simulink model "DP_STD_MDL_Boost_2022b"  (R2022b)
settings: Solver=VariableStepAuto  StartTime=0.0  StopTime=0.1  RelTol=1e-3
libraries: spsSeriesRLCBranchLib x4, spsMosfetLib x2, peripheral_utilities x2, spsCurrentMeasurementLib x1, spsSecondOrderFilterLib x1, spsVoltageMeasurementLib x1, spsControlledVoltageSourceLib x1, gmp_sil_core_pack x1, spsGroundLib x1, spspowerguiLib x1
settings Model: Creator=javnson  LastModifiedBy=javnson
settings OptimizationCC: ReuseModelBlockBuffer=on
settings RTWCC: GPUComputeCapability=5.0

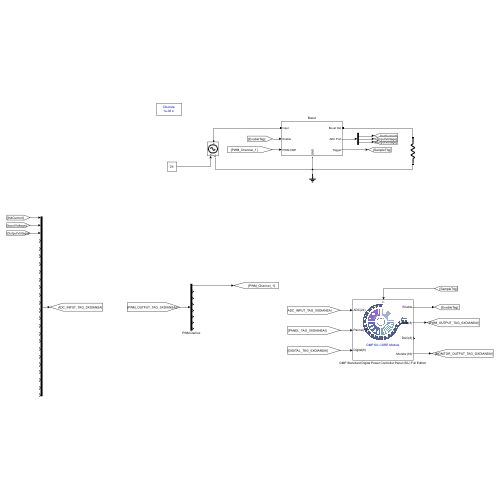
[thumbnail: Simulink's stored preview of the top-level diagram]
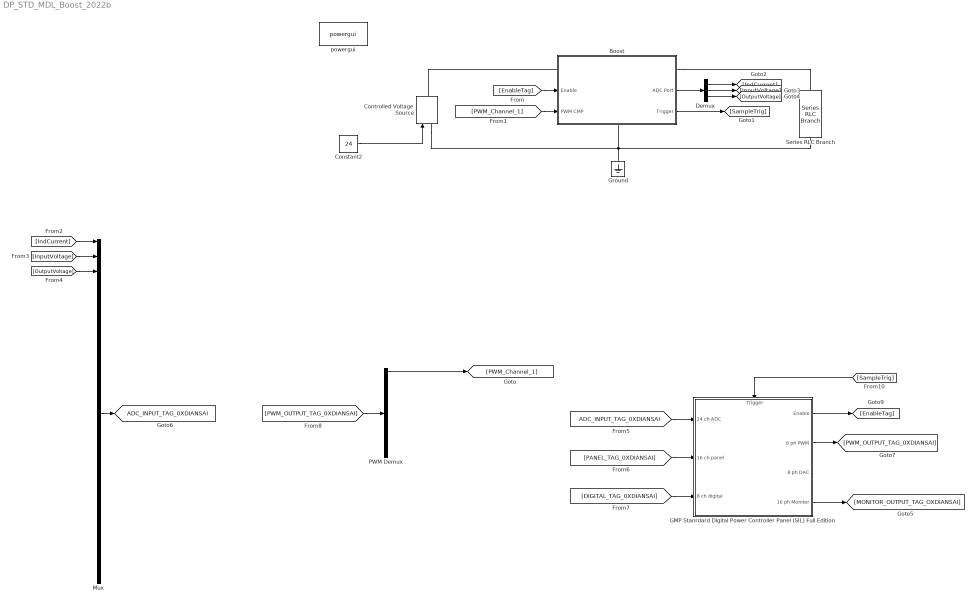
== system DP_STD_MDL_Boost_2022b ==
  Boost : Subsystem  mask(GMP Standard Digital Power Submodule - Boost){R_mosfet_on=4.6e-3, Lon=0, Rd=0.01, Vf=0.5, Rs=1e5, Cs=inf, L_main=1e-3, L_ESR=15e-3, Cin_main=100e-6, Cin_ESR=1.5, Cout_main=100e-6, Cout_ESR=1.5, fswitch=20e3, CMP_MAX=5000, Deadband_Upper=50, Deadband_Lower=50, phase_shift=0, ADC_Resolution=12, Voltage_Gain=1, VOLTAGE_ADC_REFERENCE=80, VOLTAGE_ADC_BIAS=40, VOLTAGE_ADC_INIT=0, VOLTAGE_ADC_CUT_FREQ=1.5e3, Current_Gain=1, CURRENT_ADC_REFERENCE=10, CURRENT_ADC_BIAS=5, CURRENT_ADC_INIT=0}
      mask prompts: ADC_Resolution "ADC_BIT:"; Voltage_Gain "ADC_GAIN:"; VOLTAGE_ADC_REFERENCE "ADC_REFERENCE:"; VOLTAGE_ADC_BIAS "ADC_BIAS:"; VOLTAGE_ADC_INIT "ADC_INIT:"; VOLTAGE_ADC_CUT_FREQ "cut_frequency:"; Current_Gain "ADC_GAIN:"; CURRENT_ADC_REFERENCE "ADC_REFERENCE:"; CURRENT_ADC_BIAS "ADC_BIAS:"; CURRENT_ADC_INIT "ADC_INIT:"
      mask help: This is a Standard Boost Module.
      settings: PortSchema="{\"entries\":[{\"content\":{\"sides\":[{\"content\":{\"connectorIds\":[\"LConn1\",\"In1\",\"In2\"]},\"type\":\"ConnectorPlacement.EquallySpacedRectSide\",\"uuid\":\"14f7e26c-4d08-496b-8d9c-39acdf23712e\"},{\"content\":{\"connectorIds\":[\"RConn1\",\"Out1\",\"Out2\"],\"side\":\"RIGHT\"},\"type\":\"ConnectorPlacement.EquallySpacedRectSide\",\"uuid\":\"c4fec36d-dc89-4255-810a-778c215f41bb\"},{\"content\":{\"side\":\"TOP\"},\"type\":\"ConnectorPlacement.EquallySpacedRectSide\",\"uuid\":\"1b2864bd-03e2-4902-8158-79673144629a\"},{\"content\":{\"connectorIds\":[\"RConn2\"],\"side\":\"BOTTOM\"},\"type\":\"ConnectorPlacement.EquallySpacedRectSide\",\"uuid\":\"d3456d19-e299-4c35-abfd-6fb99773e971\"}]},\"type\":\"ConnectorPlacement.EquallySpacedConnector\",\"uuid\":\"dbc738c4-c361-40e9-b3e6-9b32447065a0\"}],\"packageUris\":[\"http://schema.mathworks.com/mf0/Connector/R2020b\"],\"version\":\"1.0\"}"
      mask DialogControl ParameterGroupVar Prompt: 参数
      mask DialogControl Container4 Prompt: Component Parameters
      mask DialogControl Container7 Prompt: MOSFET
      mask DialogControl Control8 Prompt: Rds(on), unit Ohm
      mask DialogControl Control9 Prompt: Internal diode inducctance, unit H
      mask DialogControl Control10 Prompt: Internal diode resistance Rd, unit Ohm
      mask DialogControl Control11 Prompt: Internal diode forward voltage Vf, unit V
      mask DialogControl Control12 Prompt: Snubber resistance Rs, unit ohm
      mask DialogControl Control13 Prompt: Snubber Capacitance Cs, unit F
      mask DialogControl Container8 Prompt: LC Filter
      mask DialogControl Control25 Prompt: main inductance (H):
      mask DialogControl Control26 Prompt: Inductance ESR (Ohm):
      mask DialogControl Control27 Prompt: Main Input Capacitor (F):
      mask DialogControl Control28 Prompt: Input Capcitor ESR (Ohm):
      mask DialogControl Control29 Prompt: Main Output Capacitor (F):
      mask DialogControl Control30 Prompt: Output Capcitor ESR (Ohm):
      mask DialogControl Container5 Prompt: PWM Parameers
      mask DialogControl Control3 Prompt: PWM Frequency (Hz):
      mask DialogControl Control4 Prompt: Full Scale PWM Compare value:
      mask DialogControl Control6 Prompt: (whole period is 2 * CMP_MAX ticks)
      mask DialogControl Control5 Prompt: Deadband Range Set (CMP Value):
      mask DialogControl Control7 Prompt: Single side deadband time: DEADBAND_CMP/2/CMP_MAX/fswitch
      mask DialogControl Control2 Prompt: Initial Phase Shift, unit rad
      mask DialogControl Container6 Prompt: ADC Parameters
      mask DialogControl Container9 Prompt: ADC Device
      mask DialogControl Control14 Prompt: ADC resolution:
      mask DialogControl Container10 Prompt: Voltage Sensor
      mask DialogControl Control15 Prompt: ADC Voltage Gain (Scale Factor):
      mask DialogControl Control16 Prompt: ADC reference Voltage(V)
      mask DialogControl Control Prompt: ADC Bias Voltage(V)
      mask DialogControl Control18 Prompt: ADC Initial Voltage Output (V):
      mask DialogControl Control19 Prompt: Voltage Filter cut frequency (Hz):
      mask DialogControl Control20 Prompt: Generally, this value less than switch frequency / 10, greater than motor normal frequency * 3
      mask DialogControl Container11 Prompt: Current Sensor
      mask DialogControl Control21 Prompt: ADC Current Gain (Scale Factor):
      mask DialogControl Control22 Prompt: ADC reference Current(A), ADC full scale current (when gain = 1)
      mask DialogControl Control23 Prompt: ADC Bias Current(A)
      mask DialogControl Control24 Prompt: ADC initial Current Output(A)
  Constant2 : Constant  Value=24
  Controlled Voltage Source : spsControlledVoltageSourceLib/Controlled Voltage Source  Initialize=on  Source_Type=AC  Amplitude=0  Phase=0  Frequency=0  Measurements=None
  Demux : Demux  Outputs=3
  GMP Stanrdard Digital Power Controller Panel (SIL) Full Edition : Subsystem  mask(GMP SIL Core for single Motor Controller (full edition)){}
      mask help: This is GMP Motor Simulator port.
      settings: PortSchema="{\"entries\":[{\"content\":{\"sides\":[{\"content\":{\"connectorIds\":[\"In1\",\"In2\",\"In3\"]},\"type\":\"ConnectorPlacement.EquallySpacedRectSide\",\"uuid\":\"45c67bc9-9540-469a-a4ac-1e12eb9acca3\"},{\"content\":{\"connectorIds\":[\"Out1\",\"Out2\",\"Out3\",\"Out4\"],\"side\":\"RIGHT\"},\"type\":\"ConnectorPlacement.EquallySpacedRectSide\",\"uuid\":\"a17116b4-0460-48ab-8ada-a785da6c5e29\"},{\"content\":{\"connectorIds\":[\"In4\"],\"side\":\"TOP\"},\"type\":\"ConnectorPlacement.EquallySpacedRectSide\",\"uuid\":\"15623697-512e-4e4d-ab51-f53c2346fadb\"},{\"content\":{\"side\":\"BOTTOM\"},\"type\":\"ConnectorPlacement.EquallySpacedRectSide\",\"uuid\":\"47f7968c-22c1-4f3d-97d9-242e9dbf8d30\"}]},\"type\":\"ConnectorPlacement.EquallySpacedConnector\",\"uuid\":\"f369880c-e675-4c1f-982e-a4befb03f503\"}],\"packageUris\":[\"http://schema.mathworks.com/mf0/Connector/R2020b\"],\"version\":\"1.0\"}"
      mask DialogControl ParameterGroupVar Prompt: 参数
      mask Display:
      | image(append(fileparts(which('gmp_simulink_utilities.slx')),'\icon\GMP_Core.png'));
      | color('blue');
      | %text(0.3,0.3,'GMP SIL CORE Module','horizontalAlignment','left','verticalAlignment','bottom');
      | disp('\n\n\n\n\n\n\n\nGMP SIL CORE Module');
      | %text(0,0,'y=a*x^2+b','horizontalAlignment','middle', 'verticalAlignment','bottom');
      | 
      | 
      | module_pos = get_param(gcb, 'Position');
      | width = module_pos(3) - module_pos(1);
      | %rectangle('Position',[module_pos(1),module_pos(2),module_pos(3),module_pos(4)],'FaceColor','r');
      | 
      | color('Black');
      | 
      | port_label('output', 1, 'Enable');
      | port_label('output', 2, 'PWM(8)');
      | port_label('output', 3, 'DAC(8)');
      | port_label('output', 4, 'Monitor(16)');
      | 
      | port_label('input', 1, 'ADC(24)');
      | port_label('input', 2, 'Pannel(16)');
      | port_label('input', 3, 'Digital(8)');
      | port_label('input', 4, 'T');
  Ground : spsGroundLib/Ground  LConnTagsString=a
  Mux : Mux  Inputs=24
  PWM Demux : Demux  Outputs=8
  Series RLC Branch : spsSeriesRLCBranchLib/Series RLC Branch  LConnTagsString=__new0  RConnTagsString=__new0  BranchType=R  Resistance=10  Inductance=1e-3  SetiL0=off  InitialCurrent=0  Capacitance=1e-6  Setx0=off  InitialVoltage=0  Measurements=None
  powergui : spspowerguiLib/powergui  Priority=1  SimulationMode=Discrete  SampleTime=1e-6  frequency=60  Iterations=50  frequencyindice=0  Pbase=100e6  ErrMax=1e-4  UnitsV=kV  UnitsW=MW  buscounter=0  FunctionMessages=off  echomessages=off  EnableUseOfTLC=off  CurrentSourceSwitches=off  DisableSnubberDevices=off  DisableRonSwitches=off  DisableVfSwitches=off  DisplayEquations=off  AutomaticDiscreteSolvers=off  SolverType=Tustin/Backward Euler (TBE)  Interpol=off  ExternalGateDelay=off  methode=off  Ts=100  x0status=blocks  SPID=on  SwTol=0  HookPort=off  NonlinearTolerance=1e-4  nMaxIteration=100  ContinueOnMaxIteration=off  RestoreLinks=warning  ResistiveCurrentMeasurement=off  Frange=[0:2:500]  Ylog=off  Xlog=on  ShowGrid=off  save=off  variable=ZData  structure=0  ZoomFFT=off  StartTime=0.0  cycles=1  DisplayStyle=1  fundamental=60  FreqAxis=off  MaxFrequency=1000  frequencyindicesteady=1  RmsSteady=1  display=off
  tag scope: ADC_INPUT_TAG_0XDIANSAI=global
  wires:
  [PWM_Channel_1] -> Boost/2(PWM CMP)
  Boost/1(ADC Port) -> Demux/1
  Demux/2 -> [InputVoltage]
  Demux/1 -> [IndCurrent]
  Demux/3 -> [OutputVoltage]
  Constant2/1 -> Controlled Voltage Source/1
  [SampleTrig] -> GMP Stanrdard Digital Power Controller Panel (SIL) Full Edition/4(Trigger)
  GMP Stanrdard Digital Power Controller Panel (SIL) Full Edition/1(Enable) -> [EnableTag]
  [EnableTag] -> Boost/1(Enable)
  PWM Demux/1 -> [PWM_Channel_1]
  Boost/2(Trigger) -> [SampleTrig]
  [IndCurrent] -> Mux/1
  [InputVoltage] -> Mux/2
  [OutputVoltage] -> Mux/3
  Mux/1 -> [ADC_INPUT_TAG_0XDIANSAI]
  [ADC_INPUT_TAG_0XDIANSAI] -> GMP Stanrdard Digital Power Controller Panel (SIL) Full Edition/1(24 ch ADC)
  [PANEL_TAG_0XDIANSAI] -> GMP Stanrdard Digital Power Controller Panel (SIL) Full Edition/2(16 ch panel)
  [DIGITAL_TAG_0XDIANSAI] -> GMP Stanrdard Digital Power Controller Panel (SIL) Full Edition/3(8 ch digital)
  [PWM_OUTPUT_TAG_0XDIANSAI] -> PWM Demux/1
  GMP Stanrdard Digital Power Controller Panel (SIL) Full Edition/2(8 ph PWM) -> [PWM_OUTPUT_TAG_0XDIANSAI]
  GMP Stanrdard Digital Power Controller Panel (SIL) Full Edition/4(16 ph Monitor) -> [MONITOR_OUTPUT_TAG_OXDIANSAI]
  connections:
  Controlled Voltage Source/RConn1 -- Boost/LConn1
  Controlled Voltage Source/LConn1 -- Series RLC Branch/RConn1 -- Ground/LConn1 -- Boost/RConn2
  Boost/RConn1 -- Series RLC Branch/LConn1

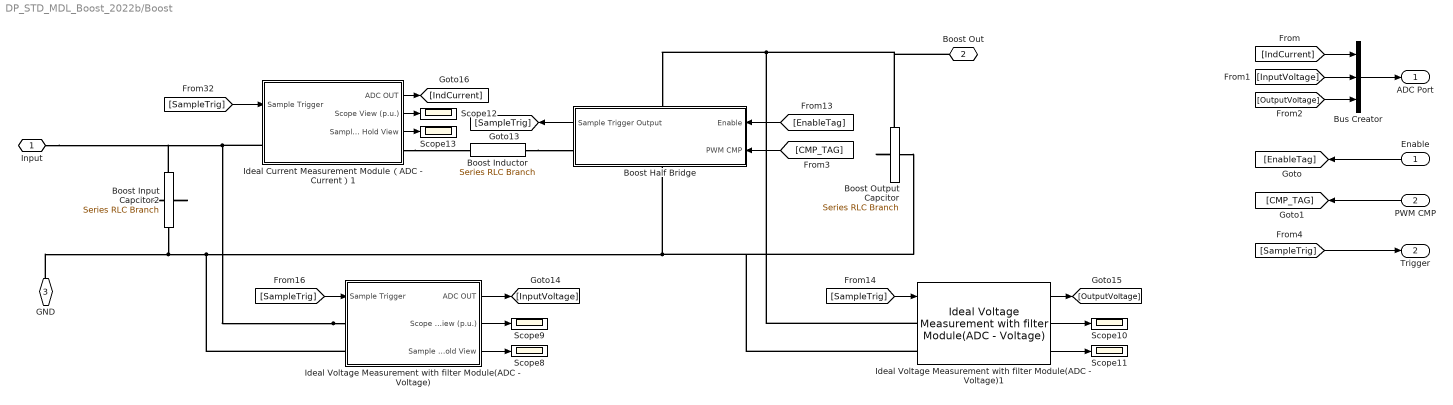
== system DP_STD_MDL_Boost_2022b/Boost ==
  Enable : Inport
  PWM CMP : Inport  Port=2
  Boost Half Bridge : Subsystem  AncestorBlock=peripheral_utilities/Single Phase Full Bridge  mask{fswitch=fswitch, CMP_MAX=CMP_MAX, Deadband_Upper=Deadband_Upper, Deadband_Lower=Deadband_Lower, Deadband_us=NaN, phase_shift=phase_shift, R_mosfet_on=R_mosfet_on, Lon=Lon, Rd=Rd, Vf=Vf, Rs=Rs, Cs=Cs}
      mask init:
      | calculate_deadband(gcb, 'Deadband_Upper', 'Deadband_Lower',	'CMP_MAX', 'fswitch', 'Deadband_us');
      settings: PortSchema="{\"entries\":[{\"content\":{\"sides\":[{\"content\":{\"connectorIds\":[\"In1\",\"In2\"]},\"type\":\"ConnectorPlacement.EquallySpacedRectSide\",\"uuid\":\"20beeabc-b0ca-4337-b227-c7f02abd15d8\"},{\"content\":{\"connectorIds\":[\"Out1\",\"RConn1\"],\"side\":\"RIGHT\"},\"type\":\"ConnectorPlacement.EquallySpacedRectSide\",\"uuid\":\"a7923383-ac55-4621-ad1d-4d067c1fb84d\"},{\"content\":{\"connectorIds\":[\"LConn1\"],\"side\":\"TOP\"},\"type\":\"ConnectorPlacement.EquallySpacedRectSide\",\"uuid\":\"661bf0ae-1c96-4de8-96aa-28c06a0a56db\"},{\"content\":{\"connectorIds\":[\"RConn2\"],\"side\":\"BOTTOM\"},\"type\":\"ConnectorPlacement.EquallySpacedRectSide\",\"uuid\":\"fc2f6321-5787-4e1a-b5a2-65ed34db36b5\"}]},\"type\":\"ConnectorPlacement.EquallySpacedConnector\",\"uuid\":\"e2219b16-0a50-43ef-8183-c55a35d5a2a0\"}],\"packageUris\":[\"http://schema.mathworks.com/mf0/Connector/R2020b\"],\"version\":\"1.0\"}"
      mask Callback fswitch: calculate_deadband(gcb, 'Deadband_Upper', 'Deadband_Lower',	'CMP_MAX', 'fswitch', 'Deadband_us');
      mask Callback CMP_MAX: calculate_deadband(gcb, 'Deadband_Upper', 'Deadband_Lower',	'CMP_MAX', 'fswitch', 'Deadband_us');
      mask Callback Deadband_Upper: calculate_deadband(gcb, 'Deadband_Upper', 'Deadband_Lower',	'CMP_MAX', 'fswitch', 'Deadband_us');
      mask Callback Deadband_Lower: calculate_deadband(gcb, 'Deadband_Upper', 'Deadband_Lower',	'CMP_MAX', 'fswitch', 'Deadband_us');
      mask DialogControl DescGroupVar Prompt: Half Bridge With PWM Module
      mask DialogControl Control14 Prompt: GMP CTL Simulink Utilities: virtual peripherals
      mask DialogControl DescTextVar Prompt: This module provide a PWM (with deadband), and a MOSFET half bridge.
      mask DialogControl Container5 Prompt: PWM Modulator
      mask DialogControl ParameterGroupVar Prompt: PWM module parameters
      mask DialogControl Control2 Prompt: PWM Frequency (Hz):
      mask DialogControl Control3 Prompt: Full Scale PWM Compare value:
      mask DialogControl Control4 Prompt: (whole period is 2 * CMP_MAX ticks)
      mask DialogControl Control5 Prompt: Deadband Range Set (CMP Value):
      mask DialogControl Control6 Prompt: Single side deadband time: DEADBAND_CMP/2/CMP_MAX/fswitch
      mask DialogControl Control15 Prompt: Calculated Deadband, us
      mask DialogControl Control13 Prompt: Initial Phase Shift, unit rad
      mask DialogControl Container6 Prompt: MOSFET
      mask DialogControl Container3 Prompt: MOSFET parameters
      mask DialogControl Control7 Prompt: Rds(on), unit Ohm
      mask DialogControl Control8 Prompt: Internal diode inducctance, unit H
      mask DialogControl Control9 Prompt: Internal diode resistance Rd, unit Ohm
      mask DialogControl Control10 Prompt: Internal diode forward voltage Vf, unit V
      mask DialogControl Control11 Prompt: Snubber resistance Rs, unit ohm
      mask DialogControl Control12 Prompt: Snubber Capacitance Cs, unit F
  Boost Inductor : spsSeriesRLCBranchLib/Series RLC Branch  LConnTagsString=__new0  RConnTagsString=__new0  BranchType=RL  Resistance=L_ESR  Inductance=L_main  SetiL0=off  InitialCurrent=0  Capacitance=1e-6  Setx0=off  InitialVoltage=0  Measurements=None
  Boost Input Capcitor2 : spsSeriesRLCBranchLib/Series RLC Branch  LConnTagsString=__new0  RConnTagsString=__new0  BranchType=RC  Resistance=Cin_ESR  Inductance=1e-3  SetiL0=off  InitialCurrent=0  Capacitance=Cin_main  Setx0=off  InitialVoltage=0  Measurements=None
  Boost Output Capcitor : spsSeriesRLCBranchLib/Series RLC Branch  LConnTagsString=__new0  RConnTagsString=__new0  BranchType=RC  Resistance=Cout_ESR  Inductance=1e-3  SetiL0=off  InitialCurrent=0  Capacitance=Cout_main  Setx0=off  InitialVoltage=0  Measurements=None
  Bus Creator : BusCreator  Inputs=3
  Ideal Current Measurement Module（ADC - Current）1 : Subsystem  AncestorBlock=peripheral_utilities/Ideal Current Measurement Module（ADC - Current）  mask{ADC_GAIN=Current_Gain, ADC_BIT=ADC_Resolution, ADC_REFERENCE=CURRENT_ADC_REFERENCE, ADC_BIAS=CURRENT_ADC_BIAS, ADC_INIT=CURRENT_ADC_INIT}
      mask DialogControl DescGroupVar Prompt: Current Sample ADC Model 1
      mask DialogControl DescTextVar Prompt: This is a ideal Current Measurement Module. This module enable a bias and a gain, and finally output a ADC result.
      mask DialogControl Control8 Prompt: ADC(p.u.) = (real_current * ADC_GAIN + ADC_BIAS)/ADC_REFERENCE
      mask DialogControl Control9 Prompt: GMP CTL Simulink Utilities: virtual peripherals
      mask DialogControl ParameterGroupVar Prompt: 参数
      mask DialogControl Control7 Prompt: ADC Current Gain (Scale Factor):
      mask DialogControl Control2 Prompt: ADC resolution:
      mask DialogControl Control4 Prompt: ADC reference Current(A), ADC full scale current (when gain = 1)
      mask DialogControl Control5 Prompt: ADC Bias Current(A)
      mask DialogControl Control6 Prompt: ADC initial Current Output(A)
  Ideal Voltage Measurement with filter Module(ADC - Voltage) : Subsystem  AncestorBlock=peripheral_utilities/Ideal Voltage Measurement with filter Module(ADC - Voltage)  mask{ADC_GAIN=Voltage_Gain, ADC_BIT=ADC_Resolution, ADC_REFERENCE=VOLTAGE_ADC_REFERENCE, ADC_BIAS=VOLTAGE_ADC_BIAS, ADC_INIT=VOLTAGE_ADC_INIT, cut_frequency=VOLTAGE_ADC_CUT_FREQ}
      mask DialogControl DescGroupVar Prompt: Voltage Sample ADC Model
      mask DialogControl DescTextVar Prompt: This is a ideal Voltage Measurement Module.
      mask DialogControl Control2 Prompt: ADC(p.u.) = (real_voltage * ADC_GAIN + ADC_BIAS)/ADC_REFERENCE
      mask DialogControl Control11 Prompt: GMP CTL Simulink Utilities: virtual peripherals
      mask DialogControl ParameterGroupVar Prompt: Parameters:
      mask DialogControl Control4 Prompt: ADC Voltage Gain (Scale Factor):
      mask DialogControl Control5 Prompt: ADC resolution:
      mask DialogControl Control6 Prompt: ADC reference Voltage(V)
      mask DialogControl Control8 Prompt: ADC Bias Voltage(V)
      mask DialogControl Control7 Prompt: ADC Initial Voltage Output (V):
      mask DialogControl Control9 Prompt: Voltage Filter cut frequency (Hz):
      mask DialogControl Control10 Prompt: Generally, this value less than switch frequency / 10, greater than motor normal frequency * 3
  Ideal Voltage Measurement with filter Module(ADC - Voltage)1 : peripheral_utilities/Ideal Voltage Measurement with filter Module(ADC - Voltage)  ADC_GAIN=Voltage_Gain  ADC_BIT=ADC_Resolution  ADC_REFERENCE=VOLTAGE_ADC_REFERENCE  ADC_BIAS=VOLTAGE_ADC_BIAS  ADC_INIT=VOLTAGE_ADC_INIT  cut_frequency=VOLTAGE_ADC_CUT_FREQ
      settings: SourceProductName=Virtual Peripheral Utilities
  Scope{8..13} (6 alike) : Scope
  Input : PMIOPort  Side=Left
  Boost Out : PMIOPort  Port=2  Side=Right
  GND : PMIOPort  Port=3  Side=Right
  ADC Port : Outport
  Trigger : Outport  Port=2
  wires:
  [SampleTrig] -> Ideal Voltage Measurement with filter Module(ADC - Voltage)/1(Sample Trigger)
  [SampleTrig] -> Ideal Voltage Measurement with filter Module(ADC - Voltage)1/1
  Ideal Voltage Measurement with filter Module(ADC - Voltage)1/2 -> Scope10/1
  [EnableTag] -> Boost Half Bridge/1(Enable)
  Ideal Current Measurement Module（ADC - Current）1/2(Scope View (p.u.)) -> Scope12/1
  Ideal Current Measurement Module（ADC - Current）1/3(Sample & Hold View) -> Scope13/1
  Boost Half Bridge/1(Sample Trigger Output) -> [SampleTrig]
  [SampleTrig] -> Ideal Current Measurement Module（ADC - Current）1/1(Sample Trigger)
  Ideal Voltage Measurement with filter Module(ADC - Voltage)/3(Sample & Hold View) -> Scope8/1
  Ideal Voltage Measurement with filter Module(ADC - Voltage)1/3 -> Scope11/1
  Ideal Voltage Measurement with filter Module(ADC - Voltage)/2(Scope View (p.u.)) -> Scope9/1
  Ideal Voltage Measurement with filter Module(ADC - Voltage)1/1 -> [OutputVoltage]
  Ideal Voltage Measurement with filter Module(ADC - Voltage)/1(ADC OUT) -> [InputVoltage]
  Ideal Current Measurement Module（ADC - Current）1/1(ADC OUT) -> [IndCurrent]
  [CMP_TAG] -> Boost Half Bridge/2(PWM CMP)
  [IndCurrent] -> Bus Creator/1
  [InputVoltage] -> Bus Creator/2
  [OutputVoltage] -> Bus Creator/3
  Bus Creator/1 -> ADC Port/1
  Enable/1 -> [EnableTag]
  PWM CMP/1 -> [CMP_TAG]
  [SampleTrig] -> Trigger/1
  connections:
  Boost Input Capcitor2/RConn1 -- Ideal Voltage Measurement with filter Module(ADC - Voltage)/LConn2 -- Ideal Voltage Measurement with filter Module(ADC - Voltage)1/LConn2 -- Boost Output Capcitor/RConn1 -- Boost Half Bridge/RConn2 -- GND/RConn1
  Ideal Voltage Measurement with filter Module(ADC - Voltage)1/LConn1 -- Boost Half Bridge/LConn1 -- Boost Output Capcitor/LConn1 -- Boost Out/RConn1
  Ideal Voltage Measurement with filter Module(ADC - Voltage)/LConn1 -- Ideal Current Measurement Module（ADC - Current）1/LConn1 -- Boost Input Capcitor2/LConn1 -- Input/RConn1
  Ideal Current Measurement Module（ADC - Current）1/RConn1 -- Boost Inductor/LConn1
  Boost Inductor/RConn1 -- Boost Half Bridge/RConn1

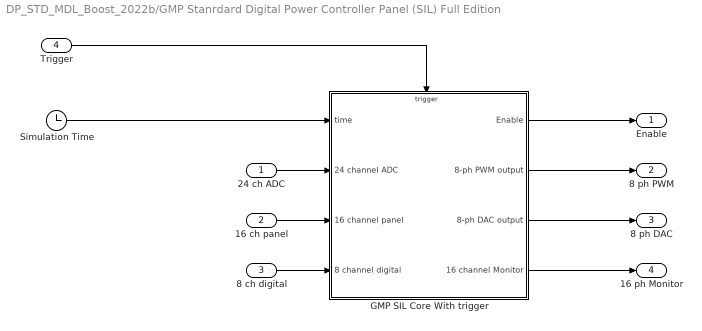
== system DP_STD_MDL_Boost_2022b/GMP Stanrdard Digital Power Controller Panel (SIL) Full Edition ==
  24 ch ADC : Inport
  16 ch panel : Inport  Port=2
  8 ch digital : Inport  Port=3
  Trigger : Inport  Port=4
  GMP SIL Core With trigger : Subsystem
  Simulation Time : Clock
  Enable : Outport
  8 ph PWM : Outport  Port=2
  8 ph DAC : Outport  Port=3
  16 ph Monitor : Outport  Port=4
  wires:
  GMP SIL Core With trigger/2(8-ph PWM output) -> 8 ph PWM/1
  Simulation Time/1 -> GMP SIL Core With trigger/1(time)
  GMP SIL Core With trigger/1(Enable) -> Enable/1
  16 ch panel/1 -> GMP SIL Core With trigger/3(16 channel panel)
  24 ch ADC/1 -> GMP SIL Core With trigger/2(24 channel ADC)
  GMP SIL Core With trigger/3(8-ph DAC output) -> 8 ph DAC/1
  Trigger/1 -> GMP SIL Core With trigger/Trigger
  8 ch digital/1 -> GMP SIL Core With trigger/4(8 channel digital)
  GMP SIL Core With trigger/4(16 channel Monitor) -> 16 ph Monitor/1

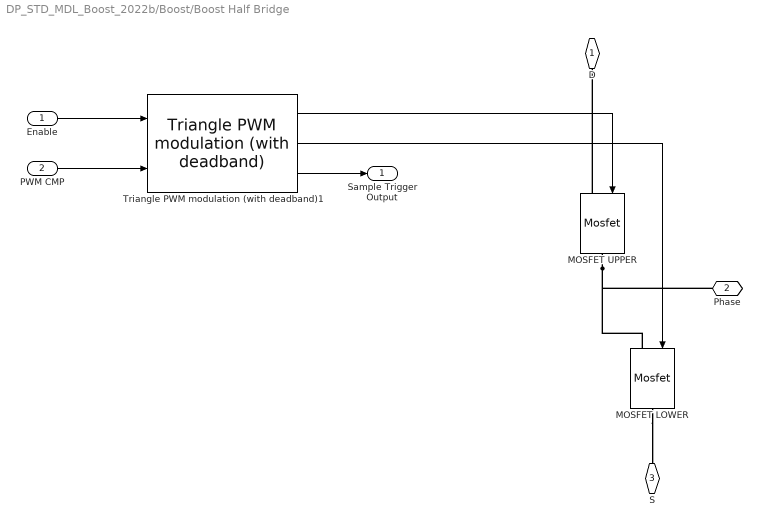
== system DP_STD_MDL_Boost_2022b/Boost/Boost Half Bridge ==
  Enable : Inport
  PWM CMP : Inport  Port=2
  MOSFET LOWER : spsMosfetLib/Mosfet  Ron=R_mosfet_on  Lon=Lon  Rd=Rd  Vfd=Vf  IC=0  Rs=Rs  Cs=Cs  Measurements=off
  MOSFET UPPER : spsMosfetLib/Mosfet  Ron=R_mosfet_on  Lon=Lon  Rd=Rd  Vfd=Vf  IC=0  Rs=Rs  Cs=Cs  Measurements=off
  Triangle PWM modulation (with deadband)1 : peripheral_utilities/Triangle PWM modulation (with deadband)  fswitch=fswitch  CMP_MAX=CMP_MAX  Deadband_Upper=Deadband_Upper  Deadband_Lower=Deadband_Lower  phase_shift=phase_shift
      settings: SourceProductName=Virtual Peripheral Utilities
  D : PMIOPort  Side=Left
  Phase : PMIOPort  Port=2  Side=Right
  S : PMIOPort  Port=3  Side=Right
  Sample Trigger Output : Outport
  wires:
  PWM CMP/1 -> Triangle PWM modulation (with deadband)1/2
  Triangle PWM modulation (with deadband)1/2 -> MOSFET LOWER/1
  Triangle PWM modulation (with deadband)1/3 -> Sample Trigger Output/1
  Enable/1 -> Triangle PWM modulation (with deadband)1/1
  Triangle PWM modulation (with deadband)1/1 -> MOSFET UPPER/1
  connections:
  MOSFET LOWER/RConn1 -- S/RConn1
  MOSFET UPPER/RConn1 -- Phase/RConn1 -- MOSFET LOWER/LConn1
  MOSFET UPPER/LConn1 -- D/RConn1

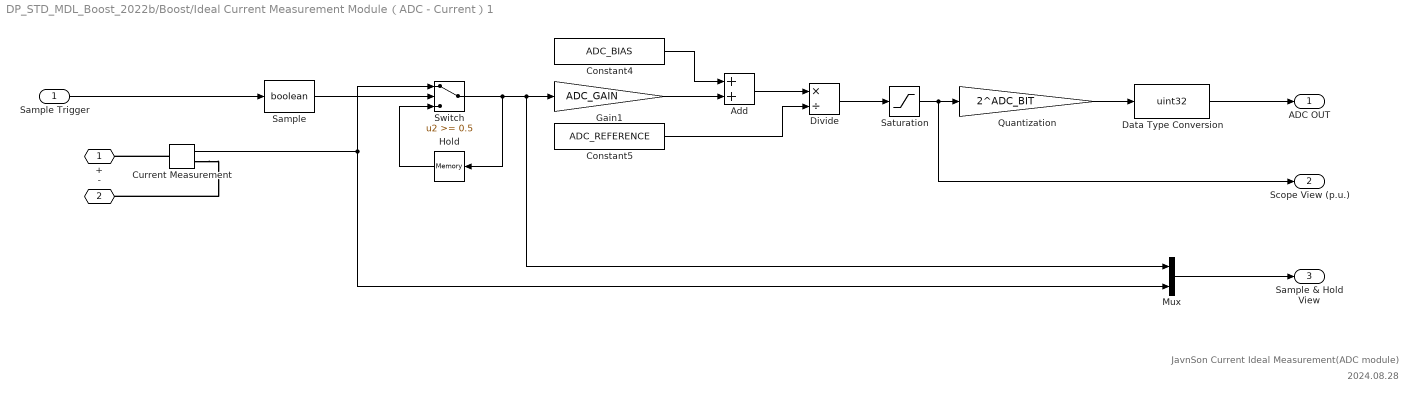
== system DP_STD_MDL_Boost_2022b/Boost/Ideal Current Measurement Module（ADC - Current）1 ==
  note: 2024.08.28
  note: JavnSon Current Ideal Measurement(ADC module)
  Sample Trigger : Inport
  Add : Sum
  Constant4 : Constant  Value=ADC_BIAS
  Constant5 : Constant  Value=ADC_REFERENCE
  Current Measurement : spsCurrentMeasurementLib/Current Measurement  PhasorSimulation=off  OutputType=Complex  PSBequivalent=0
  Data Type Conversion : DataTypeConversion  OutDataTypeStr=uint32  ConvertRealWorld=Stored Integer (SI)  SaturateOnIntegerOverflow=off  RndMeth=Floor
  Divide : Product  Inputs=*/
  Gain1 : Gain  Gain=ADC_GAIN
  Hold : Memory  InitialCondition=ADC_INIT  LinearizeAsDelay=on
  Mux : Mux  Inputs=2
  Quantization : Gain  Gain=2^ADC_BIT
  Sample : DataTypeConversion  OutDataTypeStr=boolean  SaturateOnIntegerOverflow=off  RndMeth=Floor
  Saturation : Saturate  UpperLimit=1  LowerLimit=0
  Switch : Switch  Threshold=0.5
  + : PMIOPort  Side=Left
  - : PMIOPort  Port=2  Side=Right
  ADC OUT : Outport
  Scope View (p.u.) : Outport  Port=2
  Sample & Hold View : Outport  Port=3
  wires:
  Mux/1 -> Sample & Hold View/1
  Divide/1 -> Saturation/1
  Saturation/1 -> Quantization/1, Scope View (p.u.)/1
  Gain1/1 -> Add/2
  Switch/1 -> Gain1/1, Mux/1, Hold/1
  Constant4/1 -> Add/1
  Current Measurement/1 -> Switch/1, Mux/2
  Hold/1 -> Switch/3
  Data Type Conversion/1 -> ADC OUT/1
  Sample Trigger/1 -> Sample/1
  Add/1 -> Divide/1
  Sample/1 -> Switch/2
  Quantization/1 -> Data Type Conversion/1
  Constant5/1 -> Divide/2
  connections:
  Current Measurement/RConn1 -- -/RConn1
  Current Measurement/LConn1 -- +/RConn1

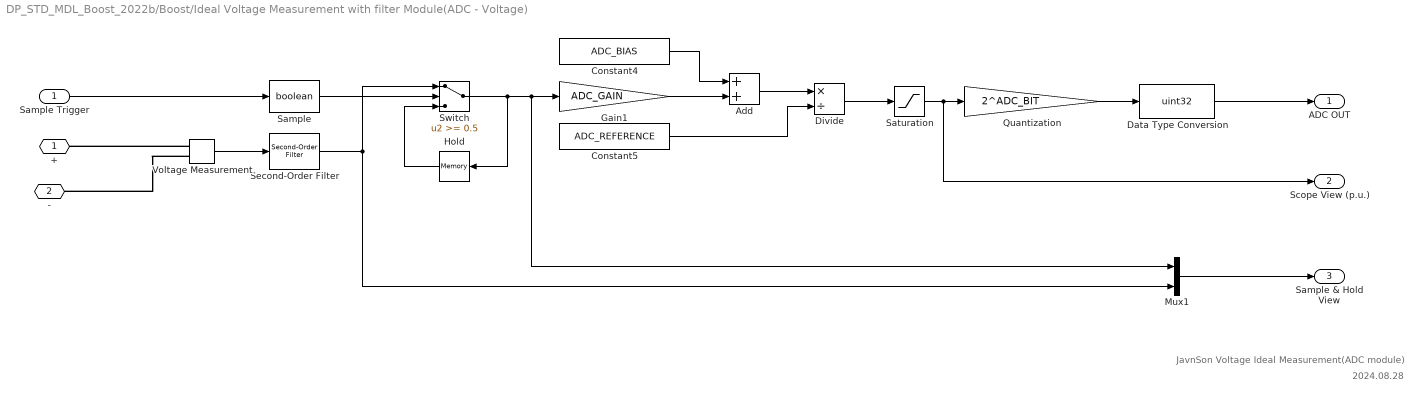
== system DP_STD_MDL_Boost_2022b/Boost/Ideal Voltage Measurement with filter Module(ADC - Voltage) ==
  note: JavnSon Voltage Ideal Measurement(ADC module)
  note: 2024.08.28
  Sample Trigger : Inport
  Add : Sum
  Constant4 : Constant  Value=ADC_BIAS
  Constant5 : Constant  Value=ADC_REFERENCE
  Data Type Conversion : DataTypeConversion  OutDataTypeStr=uint32  ConvertRealWorld=Stored Integer (SI)  SaturateOnIntegerOverflow=off  RndMeth=Floor
  Divide : Product  Inputs=*/
  Gain1 : Gain  Gain=ADC_GAIN
  Hold : Memory  InitialCondition=ADC_INIT  LinearizeAsDelay=on
  Mux1 : Mux  Inputs=2
  Quantization : Gain  Gain=2^ADC_BIT
  Sample : DataTypeConversion  OutDataTypeStr=boolean  SaturateOnIntegerOverflow=off  RndMeth=Floor
  Saturation : Saturate  UpperLimit=1  LowerLimit=0
  Second-Order Filter : spsSecondOrderFilterLib/Second-Order Filter  FilterType=Lowpass  Fo=cut_frequency  Zeta=0.707  Ts=0  Initialize=off  Vac_Init="[0,  0,  60]"  Vdc_Init=0  PlotResponse=off  FreqRange=[0, 500, 1]
  Switch : Switch  Threshold=0.5
  Voltage Measurement : spsVoltageMeasurementLib/Voltage Measurement  PhasorSimulation=off  OutputType=Complex  PSBequivalent=0
  + : PMIOPort  Side=Left
  - : PMIOPort  Port=2  Side=Left
  ADC OUT : Outport
  Scope View (p.u.) : Outport  Port=2
  Sample & Hold View : Outport  Port=3
  wires:
  Second-Order Filter/1 -> Mux1/2, Switch/1
  Hold/1 -> Switch/3
  Switch/1 -> Hold/1, Mux1/1, Gain1/1
  Divide/1 -> Saturation/1
  Voltage Measurement/1 -> Second-Order Filter/1
  Saturation/1 -> Scope View (p.u.)/1, Quantization/1
  Constant4/1 -> Add/1
  Gain1/1 -> Add/2
  Sample Trigger/1 -> Sample/1
  Data Type Conversion/1 -> ADC OUT/1
  Mux1/1 -> Sample & Hold View/1
  Quantization/1 -> Data Type Conversion/1
  Constant5/1 -> Divide/2
  Add/1 -> Divide/1
  Sample/1 -> Switch/2
  connections:
  Voltage Measurement/LConn1 -- +/RConn1
  Voltage Measurement/LConn2 -- -/RConn1

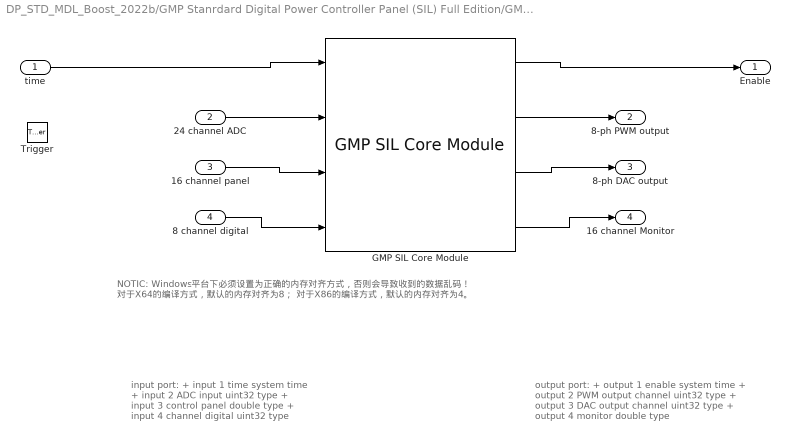
== system DP_STD_MDL_Boost_2022b/GMP Stanrdard Digital Power Controller Panel (SIL) Full Edition/GMP SIL Core With trigger ==
  note: input port:
      | + input 1 time system time
      | + input 2 ADC input uint32 type
      | + input 3 control panel double type
      | + input 4 channel digital uint32 type
  note: NOTIC:
      | Windows平台下必须设置为正确的内存对齐方式，否则会导致收到的数据乱码！
      | 对于X64的编译方式，默认的内存对齐为8；
      | 对于X86的编译方式，默认的内存对齐为4。
  note: output port:
      | + output 1 enable system time
      | + output 2 PWM output channel uint32 type
      | + output 3 DAC output channel uint32 type
      | + output 4 monitor double type
  time : Inport
  24 channel ADC : Inport  Port=2
  16 channel panel : Inport  Port=3
  8 channel digital : Inport  Port=4
  Trigger : TriggerPort  VariantControl=(inherit)  PortDimensions=1
  GMP SIL Core Module : gmp_sil_core_pack/GMP SIL Core Module  MaskPackedDataTypes={'double', 'uint32', 'double', 'int32'}  MaskPackedDataSizes={[1],[24],[16],[8]}  MaskUnpackedDataTypes={'double', 'uint32', 'uint32', 'double'}  MaskUnpackedDataSizes={[1],[8],[8],[16]}  MaskAlignment=1  MaskHostAddr='127.0.0.1'  MaskMsgTxPort=12500  MaskMsgRxPort=12501  MaskCmdTxPort=12502  MaskCmdRxPort=12503
      settings: SourceProductName=GMP SIL Core Utilities
  Enable : Outport
  8-ph PWM output : Outport  Port=2
  8-ph DAC output : Outport  Port=3
  16 channel Monitor : Outport  Port=4
  wires:
  24 channel ADC/1 -> GMP SIL Core Module/2
  16 channel panel/1 -> GMP SIL Core Module/3
  time/1 -> GMP SIL Core Module/1
  GMP SIL Core Module/3 -> 8-ph DAC output/1
  GMP SIL Core Module/2 -> 8-ph PWM output/1
  GMP SIL Core Module/1 -> Enable/1
  8 channel digital/1 -> GMP SIL Core Module/4
  GMP SIL Core Module/4 -> 16 channel Monitor/1
